simulink model "plantaCPC_2025_fuzzy_anfis"  (R2025b)
settings: Solver=ode4  StartTime=0.0  StopTime=inf  RelTol=1e-3  EnableMultiTasking=on
libraries: fuzblock x13
settings Model: PacingRate=3  Creator=Administrator  LastModifiedBy=wepi
settings SolverCC: AlgebraicLoopSolver=TrustRegion
settings DataIOCC: LimitDataPoints=on  SaveFormat=Array  ReturnWorkspaceOutputs=off
settings OptimizationCC: LifeSpan=inf
settings DebuggingCC: UnderspecifiedInitializationDetection=Classic  MergeDetectMultiDrivingBlocksExec=none  SolverPrmCheckMsg=warning  UnconnectedInputMsg=warning  UnconnectedOutputMsg=warning  UnconnectedLineMsg=warning  StateNameClashWarn=warning  SFUnexpectedBacktrackingDiag=warning  SFNoUnconditionalDefaultTransitionDiag=warning  SFExecutionAtInitializationDiag=none  ArithmeticOperatorsInVariantConditions=warning
settings HardwareCC: ProdBitPerPointer=32.0  ProdBitPerSizeT=32.0  ProdBitPerPtrDiffT=32.0  ProdLargestAtomicFloat=None  ProdIntDivRoundTo=Undefined  ProdEndianess=Unspecified  ProdWordSize=32.0  ProdHWDeviceType=32-bit Generic
settings ModelReferenceCC: PropagateSignalLabelsOutOfModel=off
settings SFSimCC: SimUseLocalCustomCode=off  CustomCodeUndefinedFunction=UseInterfaceOnly
settings RTWCC: RTWUseLocalCustomCode=off  GPUComputeCapability=3.5
settings CodeAppCC: StateflowObjectComments=on
settings GRTTargetCC: TargetLangStandard=C89/C90 (ANSI)
settings ConfigComp: CovMetricSettings=dw  CovSaveCumulativeToWorkspaceVar=on  CovSaveSingleToWorkspaceVar=on  CovExternalEMLEnable=off

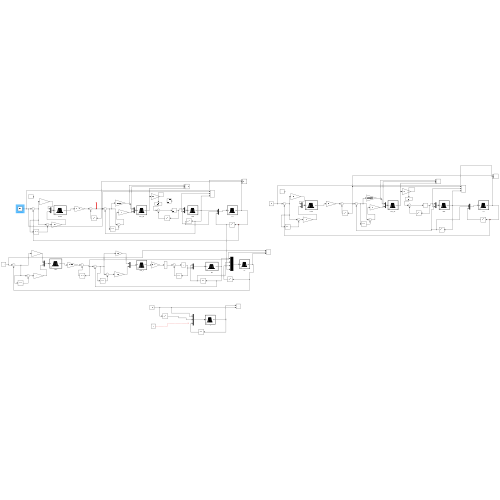
[thumbnail: Simulink's stored preview of the top-level diagram]
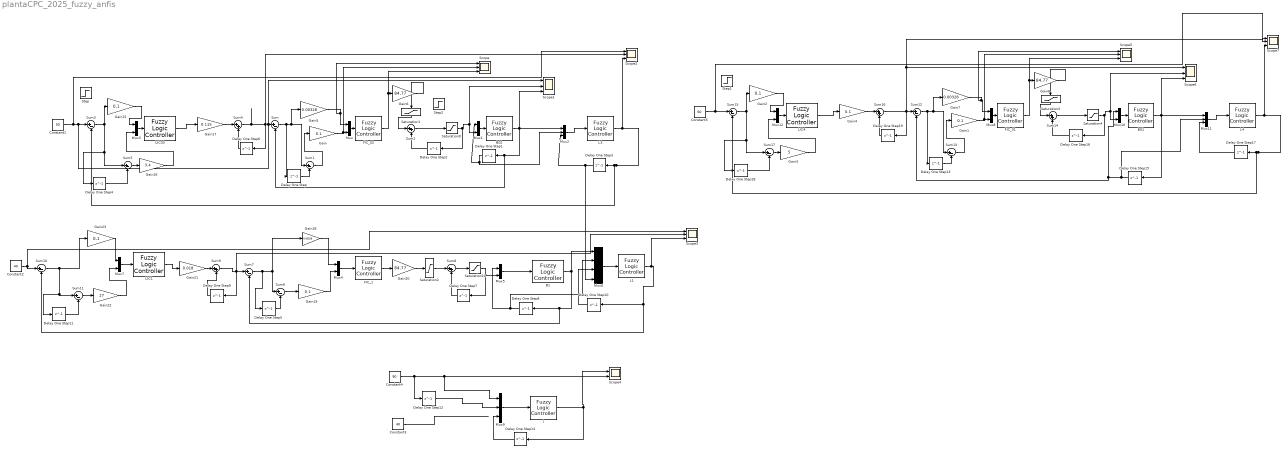
== system plantaCPC_2025_fuzzy_anfis ==
  B01 : fuzblock/Fuzzy Logic  Controller  FIS=b02  OutputSampleNumber=101  DataType=double  UseLookupTable=off  NumBreakpoints=10  FuzzifiedInputs=off  RuleFiringStrengths=off  RuleOutputs=off  AggregatedOutputs=off  SimulateUsing=Interpreted execution  OutOfRangeInputValueMessage=warning  NoRuleFiredMessage=warning  EmptyOutputFuzzySetMessage=warning
  B02 : fuzblock/Fuzzy Logic  Controller  FIS=b02  OutputSampleNumber=101  DataType=double  UseLookupTable=off  NumBreakpoints=10  FuzzifiedInputs=off  RuleFiringStrengths=off  RuleOutputs=off  AggregatedOutputs=off  SimulateUsing=Interpreted execution  OutOfRangeInputValueMessage=warning  NoRuleFiredMessage=warning  EmptyOutputFuzzySetMessage=warning
  B1 : fuzblock/Fuzzy Logic  Controller  FIS=b02  OutputSampleNumber=101  DataType=double  UseLookupTable=off  NumBreakpoints=10  FuzzifiedInputs=off  RuleFiringStrengths=off  RuleOutputs=off  AggregatedOutputs=off  SimulateUsing=Interpreted execution  OutOfRangeInputValueMessage=warning  NoRuleFiredMessage=warning  EmptyOutputFuzzySetMessage=warning
  Constant1 : Constant  Value=50
  Constant2 : Constant  Value=40
  Constant3 : Constant  Value=40
  Constant4 : Constant  Value=90
  Constant5 : Constant  Value=60
  Delay One Step{,1..19} (20 alike) : Delay  DelayLength=1  SampleTime=0.1
  FIC_01 : fuzblock/Fuzzy Logic  Controller  FIS=db  OutputSampleNumber=101  DataType=double  UseLookupTable=off  NumBreakpoints=10  FuzzifiedInputs=off  RuleFiringStrengths=off  RuleOutputs=off  AggregatedOutputs=off  SimulateUsing=Interpreted execution  OutOfRangeInputValueMessage=warning  NoRuleFiredMessage=warning  EmptyOutputFuzzySetMessage=warning
  FIC_02 : fuzblock/Fuzzy Logic  Controller  FIS=db  OutputSampleNumber=101  DataType=double  UseLookupTable=off  NumBreakpoints=10  FuzzifiedInputs=off  RuleFiringStrengths=off  RuleOutputs=off  AggregatedOutputs=off  SimulateUsing=Interpreted execution  OutOfRangeInputValueMessage=warning  NoRuleFiredMessage=warning  EmptyOutputFuzzySetMessage=warning
  FIC_1 : fuzblock/Fuzzy Logic  Controller  FIS=db  OutputSampleNumber=101  DataType=double  UseLookupTable=off  NumBreakpoints=10  FuzzifiedInputs=off  RuleFiringStrengths=off  RuleOutputs=off  AggregatedOutputs=off  SimulateUsing=Interpreted execution  OutOfRangeInputValueMessage=warning  NoRuleFiredMessage=warning  EmptyOutputFuzzySetMessage=warning
  Gain{,1..2,4,15,19,23} (7 alike) : Gain  Gain=0.1
  Gain16 : Gain  Gain=3.4
  Gain17 : Gain  Gain=0.115
  Gain18 : Gain  Gain=0.00328
  Gain20 : Gain  Gain=84.77
  Gain21 : Gain  Gain=0.018
  Gain22 : Gain  Gain=27
  Gain3 : Gain  Gain=5
  Gain5 : Gain  Gain=0.00328
  Gain6 : Gain  Gain=84.77
  Gain7 : Gain  Gain=0.00328
  Gain8 : Gain  Gain=84.77
  L1 : fuzblock/Fuzzy Logic  Controller  FIS=L1  OutputSampleNumber=101  DataType=double  UseLookupTable=off  NumBreakpoints=10  FuzzifiedInputs=off  RuleFiringStrengths=off  RuleOutputs=off  AggregatedOutputs=off  SimulateUsing=Interpreted execution  OutOfRangeInputValueMessage=warning  NoRuleFiredMessage=warning  EmptyOutputFuzzySetMessage=warning
  L3 : fuzblock/Fuzzy Logic  Controller  FIS=L3  OutputSampleNumber=101  DataType=double  UseLookupTable=off  NumBreakpoints=10  FuzzifiedInputs=off  RuleFiringStrengths=off  RuleOutputs=off  AggregatedOutputs=off  SimulateUsing=Interpreted execution  OutOfRangeInputValueMessage=warning  NoRuleFiredMessage=warning  EmptyOutputFuzzySetMessage=warning
  L4 : fuzblock/Fuzzy Logic  Controller  FIS=L4  OutputSampleNumber=101  DataType=double  UseLookupTable=off  NumBreakpoints=10  FuzzifiedInputs=off  RuleFiringStrengths=off  RuleOutputs=off  AggregatedOutputs=off  SimulateUsing=Interpreted execution  OutOfRangeInputValueMessage=warning  NoRuleFiredMessage=warning  EmptyOutputFuzzySetMessage=warning
  LIC03 : fuzblock/Fuzzy Logic  Controller  FIS=lic03  OutputSampleNumber=101  DataType=double  UseLookupTable=off  NumBreakpoints=10  FuzzifiedInputs=off  RuleFiringStrengths=off  RuleOutputs=off  AggregatedOutputs=off  SimulateUsing=Interpreted execution  OutOfRangeInputValueMessage=warning  NoRuleFiredMessage=warning  EmptyOutputFuzzySetMessage=warning
  LIC1 : fuzblock/Fuzzy Logic  Controller  FIS=lic01  OutputSampleNumber=101  DataType=double  UseLookupTable=off  NumBreakpoints=10  FuzzifiedInputs=off  RuleFiringStrengths=off  RuleOutputs=off  AggregatedOutputs=off  SimulateUsing=Interpreted execution  OutOfRangeInputValueMessage=warning  NoRuleFiredMessage=warning  EmptyOutputFuzzySetMessage=warning
  LIC4 : fuzblock/Fuzzy Logic  Controller  FIS=lic04  OutputSampleNumber=101  DataType=double  UseLookupTable=off  NumBreakpoints=10  FuzzifiedInputs=off  RuleFiringStrengths=off  RuleOutputs=off  AggregatedOutputs=off  SimulateUsing=Interpreted execution  OutOfRangeInputValueMessage=warning  NoRuleFiredMessage=warning  EmptyOutputFuzzySetMessage=warning
  Mux{,1,3..5,7..8,10,12} (9 alike) : Mux  Inputs=2
  Mux11 : Mux  Inputs=3
  Mux2 : Mux  Inputs=3
  Mux6 : Mux
  Mux9 : Mux  Inputs=3
  Saturation1 : Saturate  UpperLimit=0.2  LowerLimit=-0.2
  Saturation10 : Saturate  UpperLimit=100  LowerLimit=40
  Saturation2 : Saturate  UpperLimit=0.2  LowerLimit=-0.2
  Saturation3 : Saturate  UpperLimit=0.2  LowerLimit=-0.2
  Saturation4 : Saturate  UpperLimit=100  LowerLimit=40
  Saturation9 : Saturate  UpperLimit=100  LowerLimit=40
  Scope{,1..3,5..7} (7 alike) : Scope  NumInputPorts=3
      Scope settings: ActiveDisplayYMinimum=-0.51225332010731917  ActiveDisplayYMaximum=4.35773703556748
      Scope1 settings: ActiveDisplayYMinimum=-1.6649480645067172  ActiveDisplayYMaximum=117.58401008622187
      Scope2 settings: ActiveDisplayYMinimum=35.306583862697728  ActiveDisplayYMaximum=103.94324326954228  DataLoggingVariableName=ScopeData2
      Scope3 settings: ActiveDisplayYMinimum=-27.977118531504225  ActiveDisplayYMaximum=96.478485746927674  DataLoggingVariableName=ScopeData3
      Scope5 settings: ActiveDisplayYMinimum=-0.51225332010731917  ActiveDisplayYMaximum=4.35773703556748  DataLoggingVariableName=ScopeData5
      Scope6 settings: ActiveDisplayYMinimum=-2.256775357599345  ActiveDisplayYMaximum=86.582697954449856  DataLoggingVariableName=ScopeData6
      Scope7 settings: ActiveDisplayYMinimum=-85.443666198346023  ActiveDisplayYMaximum=246.57467457591332  DataLoggingVariableName=ScopeData7
  Scope4 : Scope  NumInputPorts=2
      settings: ActiveDisplayYMinimum=-67.849936126123936  ActiveDisplayYMaximum=128.6901245650235  DataLoggingVariableName=ScopeData4
  Step : Step  Time=40  Before=60  After=50  SampleTime=0
  Step1 : Step  Time=40  Before=60  After=50  SampleTime=0
  Step2 : Step  Time=30  Before=40  After=50  SampleTime=0
  Sum{,1,3,5..7,10..13,15,17} (12 alike) : Sum  Inputs=|+-
  Sum{2,4,8..9,14,16} (6 alike) : Sum  Inputs=|++
  l : fuzblock/Fuzzy Logic  Controller  FIS=L4  OutputSampleNumber=101  DataType=double  UseLookupTable=off  NumBreakpoints=10  FuzzifiedInputs=off  RuleFiringStrengths=off  RuleOutputs=off  AggregatedOutputs=off  SimulateUsing=Interpreted execution  OutOfRangeInputValueMessage=warning  NoRuleFiredMessage=warning  EmptyOutputFuzzySetMessage=warning
  wires:
  FIC_02/1 -> Gain6/1, Scope/3
  Sum/1 -> Sum1/1, Gain5/1, Delay One Step/1
  LIC03/1 -> Gain17/1
  Mux/1 -> FIC_02/1
  Delay One Step/1 -> Sum1/2
  Sum1/1 -> Gain/1
  Gain/1 -> Scope/2, Mux/2
  Gain5/1 -> Scope/1, Mux/1
  Saturation9/1 -> Delay One Step2/1, Mux1/2, Scope1/2
  Sum2/1 -> Saturation9/1
  B02/1 -> Scope1/3, Mux2/1, Sum/2, Delay One Step1/1
  Gain6/1 -> Saturation1/1
  Saturation1/1 -> Sum2/1
  Delay One Step2/1 -> Sum2/2
  Mux1/1 -> B02/1
  Delay One Step1/1 -> Mux1/1, Mux2/2
  Mux2/1 -> L3/1
  L3/1 -> Scope2/3, Sum3/2, Delay One Step3/1
  Delay One Step3/1 -> Mux6/4, Mux2/3
  Sum3/1 -> Sum5/1, Delay One Step4/1, Gain15/1
  Mux3/1 -> LIC03/1
  Delay One Step4/1 -> Sum5/2
  Gain15/1 -> Mux3/1
  Constant1/1 -> Scope2/1, Scope1/1, Sum/1, Sum3/1
  Gain17/1 -> Sum4/1
  Sum4/1 -> Scope2/2, Delay One Step6/1
  Delay One Step6/1 -> Sum4/2
  Gain16/1 -> Mux3/2
  Sum5/1 -> Gain16/1
  Mux4/1 -> FIC_1/1
  Gain18/1 -> Mux4/1
  Gain19/1 -> Mux4/2
  Sum6/1 -> Gain19/1
  Delay One Step5/1 -> Sum6/2
  Sum7/1 -> Delay One Step5/1, Sum6/1, Gain18/1
  FIC_1/1 -> Gain20/1
  Gain20/1 -> Saturation2/1
  Saturation2/1 -> Sum8/1
  Delay One Step7/1 -> Sum8/2
  Sum8/1 -> Saturation10/1
  Saturation10/1 -> Mux5/2, Delay One Step7/1
  Mux5/1 -> B1/1
  B1/1 -> Sum7/2, Delay One Step8/1, Mux6/1
  LIC1/1 -> Gain21/1
  Sum9/1 -> Scope3/2, Delay One Step9/1, Sum7/1
  Delay One Step8/1 -> Mux6/2, Mux5/1
  Gain21/1 -> Sum9/1
  Delay One Step9/1 -> Sum9/2
  Sum10/1 -> Delay One Step11/1, Sum11/1, Gain23/1
  Mux7/1 -> LIC1/1
  Gain23/1 -> Mux7/1
  Gain22/1 -> Mux7/2
  Sum11/1 -> Gain22/1
  Delay One Step11/1 -> Sum11/2
  Delay One Step10/1 -> Mux6/3
  Mux6/1 -> L1/1
  Constant2/1 -> Sum10/1, Scope3/1
  L1/1 -> Scope3/3, Delay One Step10/1, Sum10/2
  Mux9/1 -> l/1
  Constant4/1 -> Mux9/1, Scope4/2, Delay One Step12/1
  Delay One Step12/1 -> Mux9/2
  l/1 -> Scope4/1, Delay One Step14/1
  Constant3/1 -> ?
  Delay One Step14/1 -> Mux9/3
  LIC4/1 -> Gain4/1
  Gain8/1 -> Saturation3/1
  Mux11/1 -> L4/1
  Saturation4/1 -> Delay One Step16/1, Mux10/2, Scope6/2
  Sum16/1 -> Scope6/1, Scope7/2, Delay One Step19/1, Sum12/1
  Constant5/1 -> Scope7/1, Sum15/1
  Delay One Step19/1 -> Sum16/2
  Sum14/1 -> Saturation4/1
  FIC_01/1 -> Gain8/1, Scope5/3
  Delay One Step16/1 -> Sum14/2
  Sum15/1 -> Sum17/1, Delay One Step18/1, Gain2/1
  B01/1 -> Scope6/3, Mux11/1, Delay One Step15/1
  Gain2/1 -> Mux12/1
  Delay One Step13/1 -> Sum13/2
  L4/1 -> Scope7/3, Sum15/2, Delay One Step17/1
  Sum12/1 -> Sum13/1, Gain7/1, Delay One Step13/1
  Gain7/1 -> Scope5/1, Mux8/1
  Sum17/1 -> Gain3/1
  Delay One Step18/1 -> Sum17/2
  Gain4/1 -> Sum16/1
  Delay One Step17/1 -> Mux11/3
  Gain1/1 -> Scope5/2, Mux8/2
  Sum13/1 -> Gain1/1
  Gain3/1 -> Mux12/2
  Mux8/1 -> FIC_01/1
  Mux10/1 -> B01/1
  Delay One Step15/1 -> Mux11/2, Mux10/1, Sum12/2
  Mux12/1 -> LIC4/1
  Saturation3/1 -> Sum14/1
